simulink model "afe_dqctrl_inv_psm"  (R2026a)
settings: Solver=ode23t  StopTime=simlength  FixedStep=tc  MaxStep=glb_time.tc  RelTol=1e-4
values from neighbouring files (symbols this model uses):
  afe_ctrl = ctrl_afe_setup(glb_time.ts_afe, grid_emu.omega_grid_nom)    [init_model.m]
  afe_pwm_phase_shift_mod1 = 0    [init_model.m]
  CTRPIFF_CLIP_RELEASE = 0.001    [init_model.m]
  filters = setup_global_filters(glb_time.ts_afe, glb_time.ts_inv, glb_time.ts_dab, glb_time.tc)    [init_model.m]
  glb_time = timing_setup(fpwm_afe, trgo_afe, fpwm_inv, trgo_inv, fpwm_single_phase_inv, trgo_single_phase_inv, fpwm_dab, trgo_dab,      fpwm_psfbc, trgo_psfbc, fpwm_isop_rail, trgo_isop_rail, fpwm_cllc, trgo_cllc, t_measure, tc_factor, tc_decimation, delay_pwm, dead_time_afe,      dead_time_inv, dead_time_single_phase_inv, dead_time_dab, dead_time_psfbc, dead_time_isop_rail, dead_time_cllc)    [init_model.m]
  grid_emu = grid_three_phase_emulator('Dyn11', delta_star, grid_nominal_power, application_voltage, us1, us2, fgrid,                  eq_grid_inductance, eq_grid_resistance, eta, ucc, i1m, p_iron, n1, n2, core_area, core_length, mur,                  up_xi_pu_ref, up_eta_pu_ref, un_xi_pu_ref, un_eta_pu_ref)    [init_model.m]
  heatsink = liquid_cooled_plate_2kw_setup(weight, no_weight, cp_al, heat_capacity_hs, thermal_conductivity_al,      Rth_switch_HA, Rth_mosfet_HA, Rth_diode_HA, Tambient, DThs_init)    [init_model.m]
  inv_pwm_phase_shift_mod1 = 0    [init_model.m]
  ki_align = 18    [init_model.m]
  kp_align = 0.25    [init_model.m]
  lim_down_align = -0.05    [init_model.m]
  lim_up_align = 0.05    [init_model.m]
  omega_m_sim = psm.omega_m_bez    [init_model.m]
  psm = psm_calculus()    [init_model.m]
  psm_ctrl = ctrl_pmsm_setup(glb_time.ts_inv, psm.omega_bez, u_psm_scale, psm.Jm_norm)    [init_model.m]
  simlength = 1.75    [init_model.m]
  Tambient = 40    [init_model.m]
  time_gain_afe_module_1 = 1.0002    [init_model.m]
  time_gain_inv_module_2 = 1.001    [init_model.m]
  time_start_motor_control = 0.25    [init_model.m]
  torque_overload_factor = 1.15    [init_model.m]
  u_cm_comp_mod1 = 0    [init_model.m]
  u_psm_scale_ekf = sqrt(3)/2 * 2/3 * hwdata.inv.udc_nom/psm.ubez    [init_model.m]
undefined symbols (not defined in the file or in its folder): hwdata, igbt, magnitude, omega_m_bez, rpm_base, torque_base
libraries: fl_lib x99, nesl_utility x96, igbt_simple_lib x12, single_phase_transformer_lib x3, threephase_inductor_lib x2, dclink_for_two_levels x2, three_phase_pwm_modulator x2, cstblocks_lti x2, discrete_time_low_pass_filter x1, lithium_ion_battery x1, three_phase_voltage_with_frt_emulator x1, simple_flexible_shaft x1
(part 9 of 9)

== system afe_dqctrl_inv_psm/afe_dq_mod1/AFE_control/afe_control/grid_voltage_phase_lock_loops/FHT-PLL/pll_stageA/filter_and_transformation/FHTbeta ==
  u : Inport
  Bus Selector : BusSelector  OutputSignals=output_pu_hat,output_pu_hat_dot
  C Caller : CCaller  FunctionName=first_harmonic_tracker_process_simulink  PortSpecificationStruct="%)30     .    B \\   8    (     @         %    \"     D    !     0         %  0 \"0    $    _    07)G3F%M90  4&]R=$YA;64 4V-O<&4     26YD97@     5'EP90      4VEZ90      27-';&]B86P   X    P    !@    @    $          4    (     0    ,    !         !   P!O=70 #@   #     &    \"     0         !0    @    !     P    $         $  # &]U=  .    .     8    (    !          %    \"     $    &     0         0  ...(+4988 chars)"
  Constant : Constant  Value=glb_time.ts_afe
  Constant1 : Constant  Value=14
  Constant4 : Constant  Value=afe_ctrl.fht_grid.omega_fht
  Constant5 : Constant  Value=afe_ctrl.fht_grid.delta_fht
  Constant6 : Constant  Value=afe_ctrl.fht_grid.Ld_fht(1)
  Constant7 : Constant  Value=afe_ctrl.fht_grid.Ld_fht(2)
  Data Type Conversion{1..2,6..9} (6 alike) : DataTypeConversion  OutDataTypeStr=single  SaturateOnIntegerOverflow=off  RndMeth=Floor
  Data Type Conversion10 : DataTypeConversion  OutDataTypeStr=double  SaturateOnIntegerOverflow=off  RndMeth=Floor
  Data Type Conversion3 : DataTypeConversion  OutDataTypeStr=uint8  SaturateOnIntegerOverflow=off  RndMeth=Floor
  Data Type Conversion4 : DataTypeConversion  OutDataTypeStr=double  SaturateOnIntegerOverflow=off  RndMeth=Floor
  Data Type Conversion5 : DataTypeConversion  OutDataTypeStr=uint8  SaturateOnIntegerOverflow=off  RndMeth=Floor
  Gain : Gain  Gain=1/afe_ctrl.fht_grid.omega_fht
  Step : Step  Time=0.0125  InitialValue=1  FinalValue=0
  ud_hat : Outport
  uq_hat : Outport  Port=2
  wires:
  Gain/1 -> uq_hat/1
  Bus Selector/2 -> Data Type Conversion10/1  "<output_pu_hat_dot>"
  Data Type Conversion10/1 -> Gain/1
  Data Type Conversion4/1 -> ud_hat/1
  Data Type Conversion3/1 -> C Caller/1
  Data Type Conversion1/1 -> C Caller/3
  Data Type Conversion2/1 -> C Caller/2
  C Caller/1 -> Bus Selector/1
  Bus Selector/1 -> Data Type Conversion4/1  "<output_pu_hat>"
  Step/1 -> Data Type Conversion3/1
  u/1 -> Data Type Conversion2/1
  Constant/1 -> Data Type Conversion1/1
  Constant1/1 -> Data Type Conversion5/1
  Constant4/1 -> Data Type Conversion6/1
  Constant6/1 -> Data Type Conversion8/1
  Constant7/1 -> Data Type Conversion9/1
  Constant5/1 -> Data Type Conversion7/1
  Data Type Conversion5/1 -> C Caller/8
  Data Type Conversion6/1 -> C Caller/4
  Data Type Conversion7/1 -> C Caller/5
  Data Type Conversion8/1 -> C Caller/6
  Data Type Conversion9/1 -> C Caller/7

== system afe_dqctrl_inv_psm/afe_dq_mod1/AFE_control/afe_control/grid_voltage_phase_lock_loops/FHT-PLL_simulink/pll_stageA/filter_and_transformation/FHTalpha ==
  u : Inport
  Gain : Gain  Gain=afe_ctrl.fht_grid.Ld_fht  Multiplication=Matrix(K*u)
  Gain1 : Gain  Gain=afe_ctrl.fht_grid.Ad_fht  Multiplication=Matrix(K*u)
  Gain2 : Gain  Gain=afe_ctrl.fht_grid.Cfht  Multiplication=Matrix(K*u)
  Gain3 : Gain  Gain=1/afe_ctrl.fht_grid.omega_fht
  Selector : Selector  InputPortWidth=2  IndexOptions=Index vector (dialog)  Indices=1  OutputSizes=1
  Selector1 : Selector  InputPortWidth=2  IndexOptions=Index vector (dialog)  Indices=2  OutputSizes=1
  Sum : Sum  Inputs=-+|
  Sum1 : Sum  Inputs=|++
  Unit Delay : UnitDelay  SampleTime=-1
  ualpha : Outport
  ubeta : Outport  Port=2
  wires:
  u/1 -> Sum/2
  Unit Delay/1 -> Gain2/1, Selector1/1, Selector/1, Gain1/1
  Sum/1 -> Gain/1
  Sum1/1 -> Unit Delay/1
  Gain1/1 -> Sum1/2
  Gain2/1 -> Sum/1
  Selector/1 -> ualpha/1
  Gain/1 -> Sum1/1
  Selector1/1 -> Gain3/1
  Gain3/1 -> ubeta/1

== system afe_dqctrl_inv_psm/afe_dq_mod1/AFE_control/afe_control/grid_voltage_phase_lock_loops/FHT-PLL_simulink/pll_stageA/filter_and_transformation/FHTbeta ==
  u : Inport
  Gain : Gain  Gain=afe_ctrl.fht_grid.Ld_fht  Multiplication=Matrix(K*u)
  Gain1 : Gain  Gain=afe_ctrl.fht_grid.Ad_fht  Multiplication=Matrix(K*u)
  Gain2 : Gain  Gain=afe_ctrl.fht_grid.Cfht  Multiplication=Matrix(K*u)
  Gain3 : Gain  Gain=1/afe_ctrl.fht_grid.omega_fht
  Selector : Selector  InputPortWidth=2  IndexOptions=Index vector (dialog)  Indices=1  OutputSizes=1
  Selector1 : Selector  InputPortWidth=2  IndexOptions=Index vector (dialog)  Indices=2  OutputSizes=1
  Sum : Sum  Inputs=-+|
  Sum1 : Sum  Inputs=|++
  Unit Delay : UnitDelay  SampleTime=-1
  ualpha : Outport
  ubeta : Outport  Port=2
  wires:
  Gain3/1 -> ubeta/1
  Selector1/1 -> Gain3/1
  Gain/1 -> Sum1/1
  Selector/1 -> ualpha/1
  Gain2/1 -> Sum/1
  Gain1/1 -> Sum1/2
  Sum1/1 -> Unit Delay/1
  Sum/1 -> Gain/1
  Unit Delay/1 -> Gain1/1, Selector/1, Selector1/1, Gain2/1
  u/1 -> Sum/2

== system afe_dqctrl_inv_psm/afe_dq_mod1/AFE_control/afe_control/grid_voltage_phase_lock_loops/dq_pll/pll_stageA/sequences/alphabeta2xieta ==
  alpha : Inport
  beta : Inport  Port=2
  gamma : Inport  Port=3
  alphabeta2xieta_neg : MATLAB Function  TreatAsAtomicUnit=on
  alphabeta2xieta_pos : MATLAB Function  TreatAsAtomicUnit=on
  xi : Outport
  eta : Outport  Port=2
  Out3 : Outport  Port=3
  Out4 : Outport  Port=4
  wires:
  alpha/1 -> alphabeta2xieta_neg/1(alpha), alphabeta2xieta_pos/1(alpha)  "u_grid_alpha"
  beta/1 -> alphabeta2xieta_neg/2(beta), alphabeta2xieta_pos/2(beta)  "u_grid_beta"
  gamma/1 -> alphabeta2xieta_neg/3(gamma), alphabeta2xieta_pos/3(gamma)  "phase_grid"
  alphabeta2xieta_pos/1(xi) -> xi/1  "u_grid_pos_xi"
  alphabeta2xieta_pos/2(eta) -> eta/1  "u_grid_pos_eta"
  alphabeta2xieta_neg/1(xi) -> Out3/1  "u_grid_neg_xi"
  alphabeta2xieta_neg/2(eta) -> Out4/1  "u_grid_neg_eta"

== system afe_dqctrl_inv_psm/inv_dq_mod1/INV_control/inverter_control/current_ctrl/bemf_observer/EKF_bemf_observer/extended_kalman_observer/A_ekf ==
  Gain1 : Gain  Gain=psm_ctrl.ekf.A6_tilde_ekf
  Gain{7,9..10,13,20} (5 alike) : Gain  Gain=psm.omega_bez
  Gain{2,4,6,11,16,18} (6 alike) : Gain  Gain=glb_time.ts_inv
  Gain15 : Gain  Gain=psm_ctrl.ekf.A2_tilde_ekf
  Gain17 : Gain  Gain=psm_ctrl.ekf.A3_tilde_ekf
  Gain3 : Gain  Gain=psm_ctrl.ekf.A4_tilde_ekf
  Gain5 : Gain  Gain=psm_ctrl.ekf.A5_tilde_ekf
  I1 : Constant  Value=eye(6)
  I2 : Constant  Value=psm_ctrl.ekf.A1_tilde_ekf
  Sum7 : Sum  Inputs=+++++++
  out : Outport
  wires:
  Sum7/1 -> out/1
  I2/1 -> Gain11/1
  I1/1 -> Sum7/1
  Gain1/1 -> Gain2/1
  Gain3/1 -> Gain4/1
  Gain5/1 -> Gain6/1
  [omega_hat_kalman] -> Gain1/1
  [psi_alpha_hat] -> Gain3/1
  [psi_beta_hat] -> Gain5/1
  Gain11/1 -> Gain7/1
  Gain4/1 -> Gain9/1
  Gain6/1 -> Gain10/1
  Gain7/1 -> Sum7/2
  Gain9/1 -> Sum7/5
  Gain10/1 -> Sum7/6
  Gain18/1 -> Gain13/1
  Gain16/1 -> Gain20/1
  Gain17/1 -> Gain18/1
  Gain15/1 -> Gain16/1
  Gain13/1 -> Sum7/4
  Gain20/1 -> Sum7/3
  [i_beta_hat] -> Gain17/1
  [i_alpha_hat] -> Gain15/1
  Gain2/1 -> Sum7/7

== system afe_dqctrl_inv_psm/inv_dq_mod1/INV_control/inverter_control/current_ctrl/bemf_observer/EKF_bemf_observer/extended_kalman_observer/correlation_matrix ==
  A_ekf : Subsystem
  Gain1 : Gain  Gain=psm_ctrl.ekf.C_ekf  Multiplication=Matrix(u*K)
  Gain10 : Gain  Gain=psm_ctrl.ekf.C_ekf'  Multiplication=Matrix(u*K)
  Gain8 : Gain  Gain=psm_ctrl.ekf.C_ekf'  Multiplication=Matrix(u*K)
  Gain9 : Gain  Gain=psm_ctrl.ekf.C_ekf  Multiplication=Matrix(K*u)
  I6 : Constant  Value=eye(6)
  Product{,2,5..6} (4 alike) : Product  Multiplication=Matrix(*)
  Product3 : Product  Inputs=*/  Multiplication=Matrix(*)
  Q : Constant  Value=psm_ctrl.ekf.Qkalman
  R : Constant  Value=psm_ctrl.ekf.Rkalman
  R1 : Constant  Value=eye(2)
  Sum2 : Sum  Inputs=+-|
  Sum4 : Sum  Inputs=|++
  Sum5 : Sum  Inputs=|++
  Transpose : Math  Operator=transpose
  Unit Delay2 : UnitDelay  SampleTime=-1
  L(k) : Outport
  wires:
  A_ekf/1(out) -> Transpose/1, Product5/1
  Product6/1 -> Sum5/1
  Product3/1 -> Product/2
  Gain8/1 -> Product/1
  Sum4/1 -> Product3/2
  Sum5/1 -> Gain8/1, Gain9/1, Product2/2  "P(k|k)"
  Sum2/1 -> Product2/1
  Product/1 -> Gain1/1, L(k)/1  "L(k)"
  Gain1/1 -> Sum2/2
  R1/1 -> Product3/1
  Product2/1 -> Unit Delay2/1  "P(k+1|k)"
  Product5/1 -> Product6/1
  Gain10/1 -> Sum4/1
  Transpose/1 -> Product6/2
  R/1 -> Sum4/2
  Q/1 -> Sum5/2
  Unit Delay2/1 -> Product5/2
  Gain9/1 -> Gain10/1
  I6/1 -> Sum2/1

== system afe_dqctrl_inv_psm/inv_dq_mod1/INV_control/inverter_control/current_ctrl/bemf_observer/EKF_bemf_observer/extended_kalman_observer/double_integrator_observer ==
  phase : Inport
  Gain : Gain  Gain=psm_ctrl.di_obs.komega
  Gain1 : Gain  Gain=psm_ctrl.di_obs.ktheta
  Gain2 : Gain  Gain=psm.omega_bez
  Gain3 : Gain  Gain=1/psm.omega_bez
  Gain4 : Gain  Gain=glb_time.ts_inv
  Gain5 : Gain  Gain=glb_time.ts_inv
  Gain6 : Gain  Gain=glb_time.ts_inv
  Sum : Sum  Inputs=-+|
  Sum1 : Sum  Inputs=|++
  Sum2 : Sum  Inputs=|++
  Sum8 : Sum  Inputs=++|
  Unit Delay1 : UnitDelay  InitialCondition=pi  SampleTime=-1
  Unit Delay2 : UnitDelay  SampleTime=-1
  bounder1 : MATLAB Function  TreatAsAtomicUnit=on
  bounder2 : MATLAB Function  TreatAsAtomicUnit=on
  phase_hat : Outport  VectorParamsAs1DForOutWhenUnconnected=off
  omega_pu_hat : Outport  Port=2  VectorParamsAs1DForOutWhenUnconnected=off
  wires:
  Gain1/1 -> Gain6/1
  phase/1 -> Sum/2
  Sum8/1 -> Unit Delay1/1
  Unit Delay1/1 -> bounder2/1(u)
  Sum1/1 -> Unit Delay2/1
  Gain/1 -> Gain4/1
  Unit Delay2/1 -> omega_pu_hat/1, Sum1/2, Gain5/1
  Sum2/1 -> Sum8/2
  bounder2/1(y) -> Sum2/2, phase_hat/1, Sum/1  "phase_hat"
  bounder1/1(y) -> Gain/1, Gain1/1
  Gain2/1 -> Sum8/1
  Gain3/1 -> Sum1/1
  Gain5/1 -> Gain2/1
  Sum/1 -> bounder1/1(u)
  Gain4/1 -> Gain3/1
  Gain6/1 -> Sum2/1

== system afe_dqctrl_inv_psm/inv_dq_mod1/INV_control/inverter_control/current_ctrl/current_ctrl/dq_pi_with_vector_antiwindup mod1/dq_vector_pi/bounder1 ==
  md : Inport
  m_1 : Inport  Port=2
  m : Inport  Port=3
  Constant : Constant
  Constant1 : Constant  Value=0
  Divide : Product
  Switch : Switch  Threshold=1  SaturateOnIntegerOverflow=off  InputSameDT=off
  Switch1 : Switch  Threshold=1  SaturateOnIntegerOverflow=off  InputSameDT=off
  md_sat : Outport  VectorParamsAs1DForOutWhenUnconnected=off
  clip : Outport  Port=2  VectorParamsAs1DForOutWhenUnconnected=off
  wires:
  md/1 -> Switch1/3, Divide/2
  m_1/1 -> Divide/1
  Divide/1 -> Switch1/1
  Switch1/1 -> md_sat/1
  Switch/1 -> clip/1
  m/1 -> Switch/2, Switch1/2
  Constant/1 -> Switch/1
  Constant1/1 -> Switch/3

== system afe_dqctrl_inv_psm/inv_dq_mod1/INV_control/inverter_control/current_ctrl/current_ctrl/dq_pi_with_vector_antiwindup mod1/dq_vector_pi/bounder2 ==
  m : Inport
  m_1 : Inport  Port=2
  mq : Inport  Port=3
  Constant : Constant
  Constant1 : Constant  Value=0
  Divide : Product
  Switch : Switch  Threshold=1  SaturateOnIntegerOverflow=off  InputSameDT=off
  Switch1 : Switch  Threshold=1  SaturateOnIntegerOverflow=off  InputSameDT=off
  mq_sat : Outport  VectorParamsAs1DForOutWhenUnconnected=off
  clip : Outport  Port=2  VectorParamsAs1DForOutWhenUnconnected=off
  wires:
  Constant1/1 -> Switch/3
  Constant/1 -> Switch/1
  m/1 -> Switch1/2, Switch/2
  Switch/1 -> clip/1
  Switch1/1 -> mq_sat/1
  Divide/1 -> Switch1/1
  m_1/1 -> Divide/1
  mq/1 -> Divide/2, Switch1/3

== system afe_dqctrl_inv_psm/inv_dq_mod1/INV_control/inverter_control/current_ctrl/current_ctrl/dq_pi_with_vector_antiwindup mod1/dq_vector_pi/pi_d ==
  id_tilde : Inport
  clip : Inport  Port=2
  1/Ti : Gain  Gain=psm_ctrl.kp_i  SaturateOnIntegerOverflow=on  OutDataTypeStr=Inherit: Same as input  ParamDataTypeStr=Inherit: Same as input
  Constant : Constant  Value=0
  Sum2 : Sum  Inputs=+-  SaturateOnIntegerOverflow=on
  Sum4 : Sum  SaturateOnIntegerOverflow=on
  Sum5 : Sum  SaturateOnIntegerOverflow=on
  Switch1 : Switch  Threshold=0.5  SaturateOnIntegerOverflow=off  InputSameDT=off
  Switch2 : Switch  Threshold=0.5  SaturateOnIntegerOverflow=off  InputSameDT=off
  Unit Delay1 : UnitDelay  SampleTime=-1
  Unit Delay2 : UnitDelay  SampleTime=-1
  kp1 : Gain  Gain=CTRPIFF_CLIP_RELEASE*glb_time.ts_inv  SaturateOnIntegerOverflow=on  OutDataTypeStr=Inherit: Same as input  ParamDataTypeStr=Inherit: Same as input
  kp2 : Gain  Gain=psm_ctrl.ki_i*glb_time.ts_inv  SaturateOnIntegerOverflow=on  OutDataTypeStr=Inherit: Same as input  ParamDataTypeStr=Inherit: Same as input
  ud_out : Outport  VectorParamsAs1DForOutWhenUnconnected=off
  wires:
  id_tilde/1 -> kp2/1, 1/Ti/1
  Sum5/1 -> ud_out/1
  Switch1/1 -> Unit Delay2/1
  Sum4/1 -> Sum5/2, Switch1/3
  kp1/1 -> Sum2/2
  Sum2/1 -> Switch1/1
  Unit Delay2/1 -> Sum4/2, kp1/1, Sum2/1
  1/Ti/1 -> Sum5/1
  Switch2/1 -> Sum4/1
  kp2/1 -> Switch2/3
  clip/1 -> Unit Delay1/1
  [clip] -> Switch2/2
  [clip] -> Switch1/2
  Constant/1 -> Switch2/1
  Unit Delay1/1 -> [clip]

== system afe_dqctrl_inv_psm/inv_dq_mod1/INV_control/inverter_control/current_ctrl/current_ctrl/dq_pi_with_vector_antiwindup mod1/dq_vector_pi/pi_q ==
  iq_tilde : Inport
  clip : Inport  Port=2
  1/Ti : Gain  Gain=psm_ctrl.kp_i  SaturateOnIntegerOverflow=on  OutDataTypeStr=Inherit: Same as input  ParamDataTypeStr=Inherit: Same as input
  Constant : Constant  Value=0
  Sum2 : Sum  Inputs=+-  SaturateOnIntegerOverflow=on
  Sum4 : Sum  SaturateOnIntegerOverflow=on
  Sum5 : Sum  SaturateOnIntegerOverflow=on
  Switch1 : Switch  Threshold=0.5  SaturateOnIntegerOverflow=off  InputSameDT=off
  Switch2 : Switch  Threshold=0.5  SaturateOnIntegerOverflow=off  InputSameDT=off
  Unit Delay1 : UnitDelay  SampleTime=-1
  Unit Delay2 : UnitDelay  SampleTime=-1
  kp1 : Gain  Gain=CTRPIFF_CLIP_RELEASE*glb_time.ts_inv  SaturateOnIntegerOverflow=on  OutDataTypeStr=Inherit: Same as input  ParamDataTypeStr=Inherit: Same as input
  kp2 : Gain  Gain=psm_ctrl.ki_i*glb_time.ts_inv  SaturateOnIntegerOverflow=on  OutDataTypeStr=Inherit: Same as input  ParamDataTypeStr=Inherit: Same as input
  Vqs_out : Outport  VectorParamsAs1DForOutWhenUnconnected=off
  wires:
  Constant/1 -> Switch2/1
  [clip] -> Switch1/2
  [clip] -> Switch2/2
  clip/1 -> Unit Delay1/1
  kp2/1 -> Switch2/3
  Switch2/1 -> Sum4/1
  1/Ti/1 -> Sum5/1
  Unit Delay2/1 -> Sum2/1, kp1/1, Sum4/2
  Sum2/1 -> Switch1/1
  kp1/1 -> Sum2/2
  Sum4/1 -> Sum5/2, Switch1/3
  Switch1/1 -> Unit Delay2/1
  iq_tilde/1 -> 1/Ti/1, kp2/1
  Unit Delay1/1 -> [clip]
  Sum5/1 -> Vqs_out/1

== system afe_dqctrl_inv_psm/inv_dq_mod1/INV_control/inverter_control/current_ctrl/current_ctrl/dq_pi_with_vector_antiwindup mod1/dq_vector_pi/switch ==
  clip 1 : Inport
  clip 2 : Inport  Port=2
  Constant4 : Constant
  Constant5 : Constant  Value=0
  Sum1 : Sum  SaturateOnIntegerOverflow=on
  Switch : Switch  Threshold=0.5  SaturateOnIntegerOverflow=off  InputSameDT=off
  clip : Outport  VectorParamsAs1DForOutWhenUnconnected=off
  wires:
  Constant5/1 -> Switch/3
  Switch/1 -> clip/1
  Constant4/1 -> Switch/1
  Sum1/1 -> Switch/2
  clip 1/1 -> Sum1/1
  clip 2/1 -> Sum1/2

== system afe_dqctrl_inv_psm/inv_dq_mod1/INV_control/inverter_control/current_ctrl/current_ctrl/dq_pi_with_vector_antiwindup mod1/dq_vector_pi/vector lenght ==
  md : Inport
  mq : Inport  Port=2
  Math Function : Math  Operator=magnitude^2  SignedPower=on
  Math Function1 : Math  Operator=magnitude^2  SignedPower=on
  Math Function2 : Math  Operator=reciprocal  SignedPower=on
  Sqrt : Sqrt
  Sum5 : Sum  SaturateOnIntegerOverflow=on
  m_1 : Outport  VectorParamsAs1DForOutWhenUnconnected=off
  m : Outport  Port=2  VectorParamsAs1DForOutWhenUnconnected=off
  wires:
  Sqrt/1 -> m/1, Math Function2/1
  mq/1 -> Math Function1/1
  Math Function1/1 -> Sum5/2
  Math Function/1 -> Sum5/1
  Sum5/1 -> Sqrt/1
  Math Function2/1 -> m_1/1
  md/1 -> Math Function/1

== system afe_dqctrl_inv_psm/inv_dq_mod1/INV_control/inverter_control/current_ctrl/current_ctrl/dq_pi_with_vector_antiwindup mod1/dq_vector_pi_ccaller/Reset ==
  Step : Step  Time=0.05  InitialValue=1  FinalValue=0
  en : Outport
  wires:
  Step/1 -> en/1

== system afe_dqctrl_inv_psm/inv_dq_mod1/INV_control/inverter_control/current_ctrl/bemf_observer/EKF_bemf_observer/extended_kalman_observer/correlation_matrix/A_ekf ==
  Gain1 : Gain  Gain=psm_ctrl.ekf.A6_tilde_ekf
  Gain{7..10,13,20} (6 alike) : Gain  Gain=psm.omega_bez
  Gain{2,4,6,11,16,18} (6 alike) : Gain  Gain=glb_time.ts_inv
  Gain15 : Gain  Gain=psm_ctrl.ekf.A2_tilde_ekf
  Gain17 : Gain  Gain=psm_ctrl.ekf.A3_tilde_ekf
  Gain3 : Gain  Gain=psm_ctrl.ekf.A4_tilde_ekf
  Gain5 : Gain  Gain=psm_ctrl.ekf.A5_tilde_ekf
  I1 : Constant  Value=eye(6)
  I2 : Constant  Value=psm_ctrl.ekf.A1_tilde_ekf
  Sum7 : Sum  Inputs=+++++++
  out : Outport
  wires:
  Sum7/1 -> out/1
  I2/1 -> Gain11/1
  I1/1 -> Sum7/1
  Gain1/1 -> Gain2/1
  Gain3/1 -> Gain4/1
  Gain5/1 -> Gain6/1
  [omega_hat_kalman] -> Gain1/1
  [psi_alpha_hat] -> Gain3/1
  [psi_beta_hat] -> Gain5/1
  Gain11/1 -> Gain7/1
  Gain2/1 -> Gain8/1
  Gain4/1 -> Gain9/1
  Gain6/1 -> Gain10/1
  Gain7/1 -> Sum7/2
  Gain9/1 -> Sum7/5
  Gain10/1 -> Sum7/6
  Gain8/1 -> Sum7/7
  Gain18/1 -> Gain13/1
  Gain16/1 -> Gain20/1
  Gain17/1 -> Gain18/1
  Gain15/1 -> Gain16/1
  Gain13/1 -> Sum7/4
  Gain20/1 -> Sum7/3
  [i_beta_hat] -> Gain17/1
  [i_alpha_hat] -> Gain15/1

== matlab function afe_dqctrl_inv_psm/grid/power meter iec mfunc/three_phase_power_meter_iec ==
  data: phase input; m output Bus: PowerMeterIecBus; u_abc input; i_abc input; omega input; ts input; enable_time input
function m = three_phase_power_meter_iec(phase, u_abc, i_abc, omega, ts, enable_time)
%#codegen
% THREE_PHASE_POWER_METER_IEC
% Equivalente in singolo blocco MATLAB Function del sottosistema Simulink
% "three_phase_power_meter_iec" (libreria power_meter_iec).
%
% INGRESSI
%   phase       : angolo del PLL [rad]      (scalare)
%   u_abc       : tensioni di fase [V]      (3x1)
%   i_abc       : correnti di linea [A]     (3x1)
%   omega       : pulsazione di rete [rad/s] (scalare)
%   ts          : passo di campionamento [s]  -> parametro di maschera
%   enable_time : istante di abilitazione [s] -> parametro di maschera
%
% USCITA
%   m : struct (bus) con i campi, nello stesso ordine del Bus Creator
%       originale: Q1p, Q1n, P1n, P1p, U1n, U1p,
%                  i_act_1n, i_react_1n, i_act_1p, i_react_1p
%
% CATENA DI ELABORAZIONE (identica all'originale)
%   1) proiezione di ogni fase su cos(phase) e sin(phase), guadagno 2
%   2) media mobile dinamica su finestra pari a mezzo periodo di rete
%      (Tw = pi/|omega|), con lunghezza frazionaria interpolata
%   3) componenti simmetriche di sequenza diretta e inversa (Fortescue)
%   4) potenze attiva e reattiva per sequenza, tensioni concatenate RMS,
%      correnti attiva e reattiva per sequenza
%
% NOTE
%   - Il blocco deve girare a passo fisso ts (gli Zero-Order Hold di
%     ingresso dell'originale sono impliciti nel sample time del blocco).
%   - ts ed enable_time possono essere dichiarati come dati di scope
%     "Parameter" nel Symbols pane del MATLAB Function block, cosi'
%     risolvono direttamente sui parametri di maschera e la firma
%     esterna resta a 4 ingressi come nel blocco originale.

% ------------------------------------------------------------------
% Costanti
% ------------------------------------------------------------------
% MAVGFLT_SIZE_MAX = 17500;   % lunghezza buffer circolare (come originale)
MAVGFLT_SIZE_MAX = 2048;   % lunghezza buffer ridotto
NCH              = 12;      % canali filtrati: 6 per u_abc, 6 per i_abc

% Ordine canali:
%   1..3  ua_cos ub_cos uc_cos      7..9   ia_cos ib_cos ic_cos
%   4..6  ua_sin ub_sin uc_sin     10..12  ia_sin ib_sin ic_sin

% ------------------------------------------------------------------
% Stato persistente
% ------------------------------------------------------------------
persistent buf cb_index sample_count sum_short sum_long prev_input ...
           k_step period_held

if isempty(buf)
    buf          = zeros(NCH, MAVGFLT_SIZE_MAX);
    cb_index     = ones(NCH, 1);
    sample_count = ones(NCH, 1);
    sum_short    = zeros(NCH, 1);
    sum_long     = zeros(NCH, 1);
    prev_input   = zeros(NCH, 1);
    k_step       = 0;
    period_held  = 0;          % uscita iniziale dell'Enabled Subsystem
end

% ------------------------------------------------------------------
% Abilitazione (equivalente al blocco Step con Time = enable_time)
% ------------------------------------------------------------------
t_now  = k_step * ts;
k_step = k_step + 1;
enable = (t_now >= enable_time);

% ------------------------------------------------------------------
% Finestra di media: Enabled Subsystem 2*pi/w, alimentato da 2*|omega|.
% Quando |omega| = 0 l'Enabled Subsystem mantiene l'ultimo valore.
% ------------------------------------------------------------------
w2 = 2 * abs(omega);
if w2 > 0
    period_held = 2*pi / w2;   % = pi/|omega|, mezzo periodo di rete
end
period = period_held;

% ------------------------------------------------------------------
% Proiezione sin/cos, guadagno 2
% ------------------------------------------------------------------
c = cos(phase);
s = sin(phase);

x = zeros(NCH, 1);
x(1)  = 2 * u_abc(1) * c;   x(2)  = 2 * u_abc(2) * c;   x(3)  = 2 * u_abc(3) * c;
x(4)  = 2 * u_abc(1) * s;   x(5)  = 2 * u_abc(2) * s;   x(6)  = 2 * u_abc(3) * s;
x(7)  = 2 * i_abc(1) * c;   x(8)  = 2 * i_abc(2) * c;   x(9)  = 2 * i_abc(3) * c;
x(10) = 2 * i_abc(1) * s;   x(11) = 2 * i_abc(2) * s;   x(12) = 2 * i_abc(3) * s;

% ------------------------------------------------------------------
% Banco di 12 filtri a media mobile dinamica (dmavgflt_process)
% ------------------------------------------------------------------
y = zeros(NCH, 1);

if enable && period > 0

    desired = period / ts;
    if desired > (MAVGFLT_SIZE_MAX - 1)
        desired = MAVGFLT_SIZE_MAX - 1;
    end

    n_samples = floor(desired + 1);          % campioni che coprono il periodo
    frac      = desired + 1 - n_samples;     % parte frazionaria
    if n_samples < 1
        n_samples = 1;
    end

    for ch = 1:NCH

        ci = cb_index(ch);
        sc = sample_count(ch);

        if n_samples > sc
            % finestra in crescita: aggiungi campioni
            sum_short(ch) = sum_short(ch) + prev_input(ch);
            sum_long(ch)  = sum_long(ch)  + x(ch);
            sc = sc + 1;

        elseif n_samples < sc
            % finestra in contrazione: rimuovi i due campioni piu' vecchi
            i1 = mod(ci - 1 - sc,       MAVGFLT_SIZE_MAX) + 1;
            i2 = mod(ci - 1 - (sc - 1), MAVGFLT_SIZE_MAX) + 1;
            old_sum = buf(ch, i1) + buf(ch, i2);

            sum_short(ch) = sum_short(ch) + prev_input(ch) - old_sum;
            sum_long(ch)  = sum_long(ch)  + x(ch)          - old_sum;
            sc = sc - 1;

        else
            % finestra costante
            i1     = mod(ci - 1 - sc, MAVGFLT_SIZE_MAX) + 1;
            oldest = buf(ch, i1);

            sum_short(ch) = sum_short(ch) + prev_input(ch) - oldest;
            sum_long(ch)  = sum_long(ch)  + x(ch)          - oldest;
        end

        % aggiornamento buffer circolare
        buf(ch, ci)      = x(ch);
        cb_index(ch)     = mod(ci, MAVGFLT_SIZE_MAX) + 1;
        prev_input(ch)   = x(ch);
        sample_count(ch) = sc;

        % uscita: interpolazione lineare fra finestra corta e lunga
        if sc > 1
            avg_short = sum_short(ch) / (sc - 1);
        else
            avg_short = 0;
        end
        avg_long = sum_long(ch) / sc;

        y(ch) = avg_short * (1 - frac) + avg_long * frac;
    end
end
% se enable = false oppure period <= 0: y resta 0 e lo stato non evolve
% (comportamento identico all'originale)

ua_cos = y(1);  ub_cos = y(2);  uc_cos = y(3);
ua_sin = y(4);  ub_sin = y(5);  uc_sin = y(6);
ia_cos = y(7);  ib_cos = y(8);  ic_cos = y(9);
ia_sin = y(10); ib_sin = y(11); ic_sin = y(12);

% ------------------------------------------------------------------
% Componenti simmetriche (fasori con convenzione U = u_cos - j*u_sin)
% ------------------------------------------------------------------
sq3 = sqrt(3);

u1p_cos = (2*ua_cos - ub_cos - uc_cos - sq3*(uc_sin - ub_sin)) / 6;
u1p_sin = (2*ua_sin - ub_sin - uc_sin - sq3*(ub_cos - uc_cos)) / 6;
u1n_cos = (2*ua_cos - ub_cos - uc_cos - sq3*(ub_sin - uc_sin)) / 6;
u1n_sin = (2*ua_sin - ub_sin - uc_sin - sq3*(uc_cos - ub_cos)) / 6;

i1p_cos = (2*ia_cos - ib_cos - ic_cos - sq3*(ic_sin - ib_sin)) / 6;
i1p_sin = (2*ia_sin - ib_sin - ic_sin - sq3*(ib_cos - ic_cos)) / 6;
i1n_cos = (2*ia_cos - ib_cos - ic_cos - sq3*(ib_sin - ic_sin)) / 6;
i1n_sin = (2*ia_sin - ib_sin - ic_sin - sq3*(ic_cos - ib_cos)) / 6;

% ------------------------------------------------------------------
% Potenze per sequenza
% ------------------------------------------------------------------
P1p = 1.5 * (u1p_cos*i1p_cos + u1p_sin*i1p_sin);
Q1p = 1.5 * (u1p_cos*i1p_sin - u1p_sin*i1p_cos);
P1n = 1.5 * (u1n_cos*i1n_cos + u1n_sin*i1n_sin);
Q1n = 1.5 * (u1n_cos*i1n_sin - u1n_sin*i1n_cos);

% ------------------------------------------------------------------
% Tensioni concatenate RMS per sequenza: sqrt(3/2)*ampiezza di fase
% ------------------------------------------------------------------
U1p = sqrt(1.5 * (u1p_cos^2 + u1p_sin^2));
U1n = sqrt(1.5 * (u1n_cos^2 + u1n_sin^2));

% ------------------------------------------------------------------
% Correnti attiva e reattiva per sequenza (RMS di linea)
% La protezione contro la divisione per zero non era presente nello
% schema originale (i blocchi Divide restituivano Inf/NaN a U = 0).
% Portare U_MIN a 0 per replicare esattamente il comportamento vecchio.
% ------------------------------------------------------------------
U_MIN = 1e-9;

if U1p > U_MIN
    i_act_1p   = P1p / (sq3 * U1p);
    i_react_1p = Q1p / (sq3 * U1p);
else
    i_act_1p   = 0;
    i_react_1p = 0;
end

if U1n > U_MIN
    i_act_1n   = P1n / (sq3 * U1n);
    i_react_1n = Q1n / (sq3 * U1n);
else
    i_act_1n   = 0;
    i_react_1n = 0;
end

% ------------------------------------------------------------------
% Bus di uscita (stesso ordine dei campi dell'originale)
% ------------------------------------------------------------------
m.Q1p        = Q1p;
m.Q1n        = Q1n;
m.P1n        = P1n;
m.P1p        = P1p;
m.U1n        = U1n;
m.U1p        = U1p;
m.i_act_1n   = i_act_1n;
m.i_react_1n = i_react_1n;
m.i_act_1p   = i_act_1p;
m.i_react_1p = i_react_1p;

end

== matlab function afe_dqctrl_inv_psm/afe_dq_mod1/AFE_control/afe_control/current_ctrl/current_transformation/alphabeta2xieta ==
  data: alpha input; xi output; beta input; gamma input; eta output
function [xi,eta] = alphabeta2xieta(alpha,beta,gamma)

    xi  =  alpha*cos(gamma) + beta*sin(gamma);
    eta = -alpha*sin(gamma) + beta*cos(gamma);

end

== matlab function afe_dqctrl_inv_psm/afe_dq_mod1/AFE_control/afe_control/current_ctrl/current_transformation/uvw2alphabeta ==
  data: u input; alpha output; v input; w input; beta output
function [alpha,beta] = uvw2alphabeta(u,v,w)

alpha = 2/3*(u - 1/2*v - 1/2*w);
beta  = 2/3*(sqrt(3)/2*(v - w));

end

== matlab function afe_dqctrl_inv_psm/inv_dq_mod1/INV_control/inverter_control/encoder-sensorless-switch/MATLAB Function ==
  data: omega_ctrl output; phase_psm input; omega_obs input; phase_obs input; phase_ctrl output; omega_psm input; omega_th input
function [omega_ctrl, phase_ctrl] = switch_enc2obs(phase_psm, omega_obs, phase_obs, omega_psm, omega_th)

if abs(omega_psm) > omega_th
    omega_ctrl = omega_obs;
    phase_ctrl = phase_obs;
else
    omega_ctrl = omega_psm;
    phase_ctrl = phase_psm;
end

== matlab function afe_dqctrl_inv_psm/afe_dq_mod1/AFE_control/afe_control/current_ctrl/xi_eta_to_alpha_beta ==
  data: xi input; alpha output; eta input; phase input; beta output
function [alpha,beta] = xi_eta_to_alpha_beta(xi,eta,phase)

    alpha = xi*cos(phase) - eta*sin(phase);
    beta  = xi*sin(phase) + eta*cos(phase);

end

== matlab function afe_dqctrl_inv_psm/afe_dq_mod1/AFE_control/afe_control/grid_voltage_phase_lock_loops/FHT-PLL/pll_stageA/filter_and_transformation/abc2alphabeta ==
  data: a input; alpha output; b input; c input; beta output
function [alpha,beta] = abc2alphabeta(a,b,c)

alpha = 2/3*(a - 1/2*b - 1/2*c);
beta  = 1/sqrt(3)*(b - c);

end

== matlab function afe_dqctrl_inv_psm/afe_dq_mod1/AFE_control/afe_control/grid_voltage_phase_lock_loops/FHT-PLL/pll_stageA/sequences/alphabeta2xieta ==
  data: alpha input; xi output; beta input; gamma input; eta output
function [xi,eta] = alphabeta2xieta_pos(alpha,beta,gamma)

    xi  =  (alpha*cos(gamma) + beta*sin(gamma));
    eta = (-alpha*sin(gamma) + beta*cos(gamma));

end

== matlab function afe_dqctrl_inv_psm/afe_dq_mod1/AFE_control/afe_control/grid_voltage_phase_lock_loops/FHT-PLL/pll_stageB/bounder1 ==
  data: u input; y output
function y = bounder(u)
    y = -pi + mod(u+3*pi,2*pi);
end

== matlab function afe_dqctrl_inv_psm/afe_dq_mod1/AFE_control/afe_control/grid_voltage_phase_lock_loops/FHT-PLL/pll_stageB/double_integrator_observer/bounder1 ==
  data: u input; y output
function y = bounder(u)
    
    y = -pi + mod(u+3*pi,2*pi);
    
end

== matlab function afe_dqctrl_inv_psm/afe_dq_mod1/AFE_control/afe_control/grid_voltage_phase_lock_loops/FHT-PLL/pll_stageB/double_integrator_observer/bounder2 ==
  data: u input; y output
function y = bounder(u)
    
    y = -pi + mod(u+3*pi,2*pi);
    
end

== matlab function afe_dqctrl_inv_psm/afe_dq_mod1/AFE_control/afe_control/grid_voltage_phase_lock_loops/FHT-PLL_simulink/pll_stageA/filter_and_transformation/abc2alphabeta ==
  data: a input; alpha output; b input; c input; beta output
function [alpha,beta] = abc2alphabeta(a,b,c)

alpha = 2/3*(a - 1/2*b - 1/2*c);
beta  = 1/sqrt(3)*(b - c);

end

== matlab function afe_dqctrl_inv_psm/afe_dq_mod1/AFE_control/afe_control/grid_voltage_phase_lock_loops/FHT-PLL_simulink/pll_stageA/sequences/alphabeta2xieta ==
  data: alpha input; xi output; beta input; gamma input; eta output
function [xi,eta] = alphabeta2xieta_pos(alpha,beta,gamma)

    xi  =  (alpha*cos(gamma) + beta*sin(gamma));
    eta = (-alpha*sin(gamma) + beta*cos(gamma));

end

== matlab function afe_dqctrl_inv_psm/afe_dq_mod1/AFE_control/afe_control/grid_voltage_phase_lock_loops/FHT-PLL_simulink/pll_stageB/bounder1 ==
  data: u input; y output
function y = bounder(u)
    y = -pi + mod(u+3*pi,2*pi);
end

== matlab function afe_dqctrl_inv_psm/afe_dq_mod1/AFE_control/afe_control/grid_voltage_phase_lock_loops/FHT-PLL_simulink/pll_stageB/double_integrator_observer/bounder1 ==
  data: u input; y output
function y = bounder(u)
    
    y = -pi + mod(u+3*pi,2*pi);
    
end

== matlab function afe_dqctrl_inv_psm/afe_dq_mod1/AFE_control/afe_control/grid_voltage_phase_lock_loops/FHT-PLL_simulink/pll_stageB/double_integrator_observer/bounder2 ==
  data: u input; y output
function y = bounder(u)
    
    y = -pi + mod(u+3*pi,2*pi);
    
end

== matlab function afe_dqctrl_inv_psm/afe_dq_mod1/AFE_control/afe_control/grid_voltage_phase_lock_loops/dq_pll/pll_stageA/mormalization_and_transformation/abc2alphabeta ==
  data: a input; alpha output; b input; c input; beta output
function [alpha,beta] = abc2alphabeta(a,b,c)

alpha = 2/3*(a - 1/2*b - 1/2*c);
beta  = 1/sqrt(3)*(b - c);

end

== matlab function afe_dqctrl_inv_psm/afe_dq_mod1/AFE_control/afe_control/grid_voltage_phase_lock_loops/dq_pll/pll_stageA/sequences/alphabeta2xieta/alphabeta2xieta_neg ==
  data: alpha input; xi output; beta input; gamma input; eta output
function [xi,eta] = alphabeta2xieta_neg(alpha,beta,gamma)

    xi  = alpha*cos(gamma) - beta*sin(gamma);
    eta = alpha*sin(gamma) + beta*cos(gamma);

end

== matlab function afe_dqctrl_inv_psm/afe_dq_mod1/AFE_control/afe_control/grid_voltage_phase_lock_loops/dq_pll/pll_stageA/sequences/alphabeta2xieta/alphabeta2xieta_pos ==
  data: alpha input; xi output; beta input; gamma input; eta output
function [xi,eta] = alphabeta2xieta_pos(alpha,beta,gamma)

    xi  =  alpha*cos(gamma) + beta*sin(gamma);
    eta = -alpha*sin(gamma) + beta*cos(gamma);

end

== matlab function afe_dqctrl_inv_psm/afe_dq_mod1/AFE_control/afe_control/grid_voltage_phase_lock_loops/dq_pll/pll_stageB/bounder1 ==
  data: u input; y output
function y = bounder(u)
    y = -pi + mod(u+3*pi,2*pi);
end

== matlab function afe_dqctrl_inv_psm/afe_dq_mod1/AFE_control/afe_control/grid_voltage_phase_lock_loops/dq_pll/pll_stageB/double_integrator_observer/bounder1 ==
  data: u input; y output
function y = bounder(u)
    
    y = -pi + mod(u+3*pi,2*pi);
    
end

== matlab function afe_dqctrl_inv_psm/afe_dq_mod1/AFE_control/afe_control/grid_voltage_phase_lock_loops/dq_pll/pll_stageB/double_integrator_observer/bounder2 ==
  data: u input; y output
function y = bounder(u)
    
    y = -pi + mod(u+3*pi,2*pi);
    
end

== matlab function afe_dqctrl_inv_psm/inv_dq_mod1/INV_control/inverter_control/encoder-sensorless-switch/double_integrator_observer/bounder1 ==
  data: u input; y output
function y = bounder(u)
    y = -pi + mod(u+3*pi,2*pi);
end

== matlab function afe_dqctrl_inv_psm/inv_dq_mod1/INV_control/inverter_control/encoder-sensorless-switch/double_integrator_observer/bounder2 ==
  data: u input; y output
function y = bounder(u)
    y = -pi + mod(u+3*pi,2*pi);
end

== matlab function afe_dqctrl_inv_psm/inv_dq_mod1/INV_control/inverter_control/current_ctrl/bemf_observer/EKF_bemf_observer/extended_kalman_observer/double_integrator_observer/bounder1 ==
  data: u input; y output
function y = bounder(u)
    y = -pi + mod(u+3*pi,2*pi);
end

== matlab function afe_dqctrl_inv_psm/inv_dq_mod1/INV_control/inverter_control/current_ctrl/current_transformation/alphabeta2dq ==
  data: alpha input; d output; beta input; gamma input; q output
function [d,q] = alphabeta2dq(alpha,beta,gamma)

    d  =  alpha*cos(gamma) + beta*sin(gamma);
    q = -alpha*sin(gamma) + beta*cos(gamma);

end

== matlab function afe_dqctrl_inv_psm/inv_dq_mod1/INV_control/inverter_control/current_ctrl/current_transformation/uvw2alphabeta ==
  data: u input; alpha output; v input; w input; beta output
function [alpha,beta] = uvw2alphabeta(u,v,w)

alpha = 2/3*(u - 1/2*v - 1/2*w);
beta  = 2/3*(sqrt(3)/2*(v - w));

end

== matlab function afe_dqctrl_inv_psm/inv_dq_mod1/INV_control/inverter_control/current_ctrl/current_ctrl/output voltage transformation/dq2alphabeta ==
  data: d input; alpha output; q input; gamma input; beta output
function [alpha,beta] = dq2alphabeta(d,q,gamma)

    alpha  =  d*cos(gamma) - q*sin(gamma);
    beta = d*sin(gamma) + q*cos(gamma);

end

== matlab function afe_dqctrl_inv_psm/inv_dq_mod1/INV_control/inverter_control/current_ctrl/bemf_observer/EKF_bemf_observer/extended_kalman_observer/double_integrator_observer/bounder2 ==
  data: u input; y output
function y = bounder(u)
    y = -pi + mod(u+3*pi,2*pi);
end

== matlab function afe_dqctrl_inv_psm/inv_dq_mod1/INV_control/inverter_control/current_ctrl/bemf_observer/bemf_observer/double_integrator_observer/bounder1 ==
  data: u input; y output
function y = bounder(u)
    
    y = -pi + mod(u+3*pi,2*pi);
end

== matlab function afe_dqctrl_inv_psm/inv_dq_mod1/INV_control/inverter_control/current_ctrl/bemf_observer/bemf_observer/double_integrator_observer/bounder2 ==
  data: u input; y output
function y = bounder(u)
    
    u = -pi + mod(u+3*pi,2*pi);
    
    y = u;
end
